simulink model "UAV_SENSORS_IMU_GPS_PWM"  (Simulink 7.0)
settings: Solver=FixedStepDiscrete  SolverMode=SingleTasking  StartTime=0.0  StopTime=10.0  FixedStep=0.01  RelTol=1e-3
undefined symbols (not defined in the file or in its folder): getGpsMainData, Init_onlyOnce, Init_Reset, sensorMCUInit, y1
libraries: dsPICdrivers x15, simulink x1
settings Model: Creator=Lubin  LastModifiedBy=Admin
settings OptimizationCC: InlineParams=on  OptimizeModelRefInitCode=on  LifeSpan=1
settings DebuggingCC: SaveWithParameterizedLinksMsg=none  SignalResolutionControl=TryResolveAllWithWarning
settings HardwareCC: ProdBitPerInt=16  ProdEndianess=LittleEndian  ProdWordSize=16  ProdHWDeviceType=16-bit Generic  TargetHWDeviceType=32-bit Generic
settings RTWCC: SystemTargetFile=dspic.tlc  MakeCommand=make_CreateMPLAB  TemplateMakefile=dspic_pic30_gcc.tmf  PostCodeGenCommand=dsPIC_Compile()  Description=Embedded Target for Microchip dsPIC (real-time)  ProcessScript=dspic_make_rtw_hook  CustomHeaderCode="#include \"apDefinitions.h\""  CustomInclude=\mavlink\include\slugs\
settings RTWCC: CustomSource=|
  | clib\circBuffer.c
  | clib\sbrk.c
  | clib\gps.c
  | clib\interProcCommMaster.c
  | clib\mavlinkSensorMcu.c
settings CodeAppCC: IgnoreCustomStorageClasses=off
settings STFCustomTargetCC: TargetFcnLib=ansi_tfl_tmw.mat  GenFloatMathFcnCalls=ANSI_C  IncludeMdlTerminateFcn=off  CombineOutputUpdateFcns=on  SuppressErrorStatus=on  ERTCustomFileBanners=on  SupportAbsoluteTime=off  SupportNonFinite=off  SupportComplex=off  SupportContinuousTime=off  SupportNonInlinedSFcns=off  ModelStepFunctionPrototypeControlCompliant=on  SystemTargetFile=dspic.tlc
settings ERTTargetCC: TargetFcnLib=ansi_tfl_tmw.mat  GenFloatMathFcnCalls=ANSI_C  CompOptLevelCompliant=off  IncludeMdlTerminateFcn=off  SuppressErrorStatus=on  SupportAbsoluteTime=off  SupportNonFinite=off  SupportComplex=off  ExtModeMexFile=ext_serial_win32_comm  InlinedParameterPlacement=NonHierarchical  ERTSrcFileBannerTemplate=dsPIC_code_template.cgt  ERTHdrFileBannerTemplate=dsPIC_code_template.cgt  ERTDataSrcFileTemplate=dsPIC_code_template.cgt  ERTDataHdrFileTemplate=dsPIC_code_template.cgt  ERTCustomFileTemplate=dsPIC_main.tlc
settings CustomProperty: DataType=string  Value=C:\PROGRA~1\MATLAB\R2007b\bin\win32\gmake

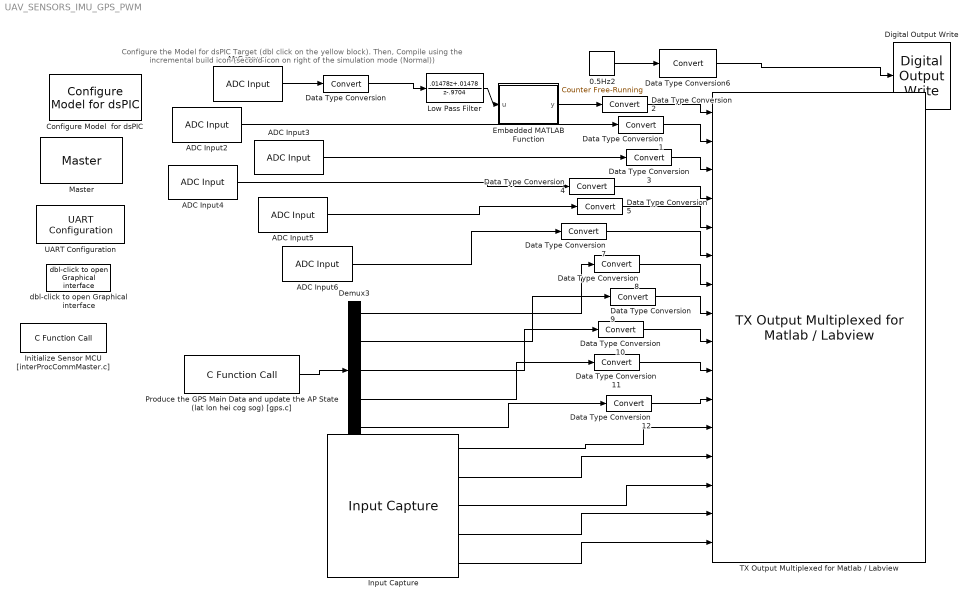
== system UAV_SENSORS_IMU_GPS_PWM ==
  note: Configure the Model for dsPIC Target (dbl click on the yellow block).
      | Then, Compile using the incremental build icon
      | (second icon on right of the simulation mode (Normal))
  0.5Hz2 : simulink/Sources/Counter Free-Running  SystemSampleTime=-1  NumBits=1  tsamp=0.5
  ADC Input1 : dsPICdrivers/Peripheral I//O/ADC Input  Tag=dsPIC_ADC  Priority=5  ADC_TYPE=12 bits  ADC_MODE=Continuous sampling & get last channel value  NbrSampleStep=1  VoltRefpopup="AVdd  -  AVss"  OutFormatBitspopup=0000 dddd dddd dddd : Integer  InterruptPriority=6  ANCHANNELS=[3]  MaxName=ANmax = 4095  Rin=5e6  ADCS=53  SAMC=31  Temperature=25  DMAChannel=0  SampleTime=.1  Status="OK  |  Tsmp=2.093e-005 |  T/Channel=3.038e-005 |  Tall=3.038e-005"  SSRC=auto convert
  ADC Input2 : dsPICdrivers/Peripheral I//O/ADC Input  Tag=dsPIC_ADC  Priority=5  ADC_TYPE=12 bits  ADC_MODE=Continuous sampling & get last channel value  NbrSampleStep=1  VoltRefpopup="AVdd  -  AVss"  OutFormatBitspopup=0000 dddd dddd dddd : Integer  InterruptPriority=6  ANCHANNELS=[4]  MaxName=ANmax = 4095  Rin=5e6  ADCS=53  SAMC=31  Temperature=25  DMAChannel=0  SampleTime=.1  Status="OK  |  Tsmp=2.093e-005 |  T/Channel=3.038e-005 |  Tall=3.038e-005"  SSRC=auto convert
  ADC Input3 : dsPICdrivers/Peripheral I//O/ADC Input  Tag=dsPIC_ADC  Priority=5  ADC_TYPE=12 bits  ADC_MODE=Continuous sampling & get last channel value  NbrSampleStep=1  VoltRefpopup="AVdd  -  AVss"  OutFormatBitspopup=0000 dddd dddd dddd : Integer  InterruptPriority=6  ANCHANNELS=[9]  MaxName=ANmax = 4095  Rin=5e6  ADCS=53  SAMC=31  Temperature=25  DMAChannel=0  SampleTime=.1  Status="OK  |  Tsmp=2.093e-005 |  T/Channel=3.038e-005 |  Tall=3.038e-005"  SSRC=auto convert
  ADC Input4 : dsPICdrivers/Peripheral I//O/ADC Input  Tag=dsPIC_ADC  Priority=5  ADC_TYPE=12 bits  ADC_MODE=Continuous sampling & get last channel value  NbrSampleStep=1  VoltRefpopup="AVdd  -  AVss"  OutFormatBitspopup=0000 dddd dddd dddd : Integer  InterruptPriority=6  ANCHANNELS=[11]  MaxName=ANmax = 4095  Rin=5e6  ADCS=53  SAMC=31  Temperature=25  DMAChannel=0  SampleTime=.1  Status="OK  |  Tsmp=2.093e-005 |  T/Channel=3.038e-005 |  Tall=3.038e-005"  SSRC=auto convert
  ADC Input5 : dsPICdrivers/Peripheral I//O/ADC Input  Tag=dsPIC_ADC  Priority=5  ADC_TYPE=12 bits  ADC_MODE=Continuous sampling & get last channel value  NbrSampleStep=1  VoltRefpopup="AVdd  -  AVss"  OutFormatBitspopup=0000 dddd dddd dddd : Integer  InterruptPriority=6  ANCHANNELS=[12]  MaxName=ANmax = 4095  Rin=5e6  ADCS=53  SAMC=31  Temperature=25  DMAChannel=0  SampleTime=.1  Status="OK  |  Tsmp=2.093e-005 |  T/Channel=3.038e-005 |  Tall=3.038e-005"  SSRC=auto convert
  ADC Input6 : dsPICdrivers/Peripheral I//O/ADC Input  Tag=dsPIC_ADC  Priority=5  ADC_TYPE=12 bits  ADC_MODE=Continuous sampling & get last channel value  NbrSampleStep=1  VoltRefpopup="AVdd  -  AVss"  OutFormatBitspopup=0000 dddd dddd dddd : Integer  InterruptPriority=6  ANCHANNELS=[15]  MaxName=ANmax = 4095  Rin=5e6  ADCS=53  SAMC=31  Temperature=25  DMAChannel=0  SampleTime=.1  Status="OK  |  Tsmp=2.093e-005 |  T/Channel=3.038e-005 |  Tall=3.038e-005"  SSRC=auto convert
  Configure Model  for dsPIC : dsPICdrivers/Simulink Configuration/Configure Model  for dsPIC
  Data Type Conversion : DataTypeConversion  OutDataTypeMode=double  OutDataType=sfix(16)  OutScaling=2^0
  Data Type Conversion{1..5,7..12} (11 alike) : DataTypeConversion  OutDataTypeMode=uint16  OutDataType=sfix(16)  OutScaling=2^0
  Data Type Conversion6 : DataTypeConversion  OutDataTypeMode=boolean  OutDataType=sfix(16)  OutScaling=2^0
  Demux3 : Demux  Outputs=5
  Digital Output Write : dsPICdrivers/Digital I//O/Digital Output Write  Tag=dsPIC_Digital_Output  Priority=5  PORT=A  Pin=[2]  Simultaneous=off  OrderingInOutPopup=None
  Embedded MATLAB Function : Stateflow chart
  Initialize Sensor MCU [interProcCommMaster.c] : dsPICdrivers/OTHERS/C Function Call  Tag=dsPIC_dsPIC_CFunctionCall  FctUpdate=Output Function  fctName='sensorMCUInit'  INPUT_SIZE=1  INPUT1=--  INPUT2=--  INPUT3=--  OUTPUT_SIZE=1  OUTPUT1=--  SampleTime=inf  InputType=[ ]  OutputType=[ ]  FctDeclaration=extern void sensorMCUInit();  FctCall=sensorMCUInit();  OrderingInOutPopup=None  FctStart=None  FctStart_Name=Init_onlyOnce  FctStart_Declaration=inline extern void Init_onlyOnce();  FctStart_Call=Init_onlyOnce();  FctInit=None  FctInit_Name=Init_Reset  FctInit_Declaration=inline extern void Init_Reset();  FctInit_Call=Init_Reset();
  Input Capture : dsPICdrivers/Peripheral I//O/Input Capture  Tag=dsPIC_PWM_IC  Priority=5  IntPriority=6  Channel=[ 2 3 4 5 8]  Channel_UP_Down_Periode="[1  1  1  1  1]"  MaxChannel="[0.0025      0.0025      0.0025      0.0025      0.0025]"  SafeMarge="[10  10  10  10  10]"  MaxName=' IC2max , IC3max , IC4max , IC5max , IC8max '  Precision="[13.7469      13.7469      13.7469      13.7469      13.7469]"  Timer="[2  2  2  2  2]"  ChangeDetected="[0  0  0  0  0]"  ChangeDetectedPortRef=3  SampleTime=.01  Status=OK
  Low Pass Filter : DiscreteTransferFcn  Numerator=[.01478 .01478]  Denominator=[1 -.9704]  SampleTime=.01
  Master : dsPICdrivers/Master  Tag=dsPIC_MASTER  Priority=1  TimeStepType=Timer1  picType=33fJ256MC710  fcy=40000000  Quartz_33f=4e6  PLLActive_33f=on  fcyDesired_33f=40e6  tmr1="[8  49999  0]"  tmr1Info="Time Step : 0.01  ;   Error : 0%  PR1=49999"  tmr2345="[1  0  0  0  0  0  0  0]"  tmr2345cfg=[-1 -1 -1 -1 -1 -1 -1 -1]  IOautoConf=on  typePort="[ 0   0  10   0   0   0   0   0   0   0   0   0   0   0   0   0   0   0   0   8   8   0   0   0   0   8   0   8   8   0   0   8   0   0   0   0   0   0   0   0   0   0   0   0   0   0   0   0   0   0   0   0   0   0   0   0   6   6   6   6   0   0   0   0   0   0   0   0   0   0   0   0   0   0   0   0   0   0   0   0   0   0   0   0   4   5   0   0   0   0   0   0   0   0   0   0   0   0   0   0   0   0   0   0   0   0   0   0   0   0   0   0 ]"  TRIS="[ 65531  65535  65535  65535  65535  65535  65535 ]"  ADPCFG=0  MasterBusyPort=None  MasterOverloadPort=None  FOSC=Quartz (XT - HS)  ClockSwitchMonitor=Both disabled  TempProtection_33f=TEMP_ON  FPBOR=<empty>  PWRT=64ms  MCLR=<empty>  ICD=ICS_PGD1  JTAGEN=JTAGEN_OFF  PowerSave=off  OverrideFcy=off  NewFcy=1e6  PR2345="[65535  65535  65535  65535  65535  65535  65535  65535]"
  Produce the GPS Main Data and update the AP State (lat lon hei cog sog) [gps.c] : dsPICdrivers/OTHERS/C Function Call  Tag=dsPIC_dsPIC_CFunctionCall  FctUpdate=Output Function  fctName='getGpsMainData'  INPUT_SIZE=1  INPUT1=--  INPUT2=--  INPUT3=--  OUTPUT_SIZE=5  OUTPUT1=real32  SampleTime=.01  InputType=[ ]  OutputType=[ 7 ]  FctDeclaration=extern void getGpsMainData(real32_T* y1);  FctCall=getGpsMainData(*%y1);  OrderingInOutPopup=None  FctStart=None  FctStart_Name=Init_onlyOnce  FctStart_Declaration=inline extern void Init_onlyOnce();  FctStart_Call=Init_onlyOnce();  FctInit=None  FctInit_Name=Init_Reset  FctInit_Declaration=inline extern void Init_Reset();  FctInit_Call=Init_Reset();
  TX Output Multiplexed for Matlab / Labview : dsPICdrivers/Serial PORT/TX Output Multiplexed for Matlab // Labview  Tag=dsPIC_TX_Multiplexed  Priority=5  UART=2  CleverSpreadingChk=on  CleverSpreading=1  CHANNEL="[0 1 2  3  4  5 6 7 8 9 10 11 12 13 14  15]"  CHANNELBLOCKED=[]  CHANNELBLOCKED_BITEWISE=0  Status=OK
  UART Configuration : dsPICdrivers/Serial PORT/UART Configuration  Tag=dsPIC_config_UART  Priority=2  UART=2  proposed_BAUD=115200  BAUD=115200  ALT_TX_RX=on  InterruptTxWhen=When Transmit Buffer is empty  TXInterruptPri=1  TxBufferSize=32  TXEN=on  InterruptRxWhen=When Receive Buffer is full (contain 4 characters)  RXInterruptPri=1  RxBufferSize=32  DoNotImplementRxInterrupt=off  DoNotImplementTxInterrupt=off  UxBRG=21  Info="UxBRG = 21   ||  Real Baud : 113636   ||  % error : -1.3573  ||  max 113.6364 Bytes / Step"  RealBaud=0  ERROR=-1.3573  BYTES_STEP=113.6364
  dbl-click to open Graphical interface : dsPICdrivers/Serial PORT/dbl-click to open Graphical interface  Nothing=0
  wires:
  0.5Hz2/1 -> Data Type Conversion6/1
  Data Type Conversion6/1 -> Digital Output Write/1
  ADC Input2/1 -> Data Type Conversion1/1
  ADC Input3/1 -> Data Type Conversion3/1
  ADC Input4/1 -> Data Type Conversion4/1
  ADC Input5/1 -> Data Type Conversion5/1
  ADC Input6/1 -> Data Type Conversion7/1
  Produce the GPS Main Data and update the AP State (lat lon hei cog sog) [gps.c]/1 -> Demux3/1
  Demux3/1 -> Data Type Conversion8/1
  Demux3/2 -> Data Type Conversion9/1
  Demux3/3 -> Data Type Conversion10/1
  Demux3/4 -> Data Type Conversion11/1
  Demux3/5 -> Data Type Conversion12/1
  Data Type Conversion2/1 -> TX Output Multiplexed for Matlab / Labview/1
  Data Type Conversion1/1 -> TX Output Multiplexed for Matlab / Labview/2
  Data Type Conversion3/1 -> TX Output Multiplexed for Matlab / Labview/3
  Data Type Conversion4/1 -> TX Output Multiplexed for Matlab / Labview/4
  Data Type Conversion5/1 -> TX Output Multiplexed for Matlab / Labview/5
  Data Type Conversion7/1 -> TX Output Multiplexed for Matlab / Labview/6
  Data Type Conversion8/1 -> TX Output Multiplexed for Matlab / Labview/7
  Data Type Conversion9/1 -> TX Output Multiplexed for Matlab / Labview/8
  Data Type Conversion10/1 -> TX Output Multiplexed for Matlab / Labview/9
  Data Type Conversion11/1 -> TX Output Multiplexed for Matlab / Labview/10
  Data Type Conversion12/1 -> TX Output Multiplexed for Matlab / Labview/11
  ADC Input1/1 -> Data Type Conversion/1
  Low Pass Filter/1 -> Embedded MATLAB Function/1(u)
  Data Type Conversion/1 -> Low Pass Filter/1
  Embedded MATLAB Function/1(y) -> Data Type Conversion2/1
  Input Capture/1 -> TX Output Multiplexed for Matlab / Labview/12
  Input Capture/2 -> TX Output Multiplexed for Matlab / Labview/13
  Input Capture/3 -> TX Output Multiplexed for Matlab / Labview/14
  Input Capture/4 -> TX Output Multiplexed for Matlab / Labview/15
  Input Capture/5 -> TX Output Multiplexed for Matlab / Labview/16

== matlab function Embedded MATLAB Function ==
  data: u input inherited; y output inherited
function y = fcn(u)
% This block supports the Embedded MATLAB subset.
% See the help menu for details. 
A=3.3/2^12;
y = u*A;
end
